simulink model "pfb_fft_d3a"  (R2021a)
settings: Solver=VariableStepAuto  StartTime=0.0  StopTime=100.0  RelTol=1e-3
undefined symbols (not defined in the file): i, pfb_coeff_gen_calc
libraries: xbsIndex_r4 x11529, casper_library_misc x39, casper_library_delays x39, xbsReplacements_r4 x2
(part 3 of 118)

== system pfb_fft_d3a/fft_wideband_real/del_4x_pol0 ==
  d : Inport
  q : Outport  VectorParamsAs1DForOutWhenUnconnected=off
  wires:
  d/1 -> q/1

== system pfb_fft_d3a/fft_wideband_real/del_4x_pol1 ==
  d : Inport
  q : Outport  VectorParamsAs1DForOutWhenUnconnected=off
  wires:
  d/1 -> q/1

== system pfb_fft_d3a/fft_wideband_real/del_4x_pol2 ==
  d : Inport
  q : Outport  VectorParamsAs1DForOutWhenUnconnected=off
  wires:
  d/1 -> q/1

== system pfb_fft_d3a/fft_wideband_real/del_4x_pol3 ==
  d : Inport
  q : Outport  VectorParamsAs1DForOutWhenUnconnected=off
  wires:
  d/1 -> q/1

== system pfb_fft_d3a/fft_wideband_real/del_4x_pol4 ==
  d : Inport
  q : Outport  VectorParamsAs1DForOutWhenUnconnected=off
  wires:
  d/1 -> q/1

== system pfb_fft_d3a/fft_wideband_real/del_4x_pol5 ==
  d : Inport
  q : Outport  VectorParamsAs1DForOutWhenUnconnected=off
  wires:
  d/1 -> q/1

== system pfb_fft_d3a/fft_wideband_real/del_4x_pol6 ==
  d : Inport
  q : Outport  VectorParamsAs1DForOutWhenUnconnected=off
  wires:
  d/1 -> q/1

== system pfb_fft_d3a/fft_wideband_real/del_4x_pol7 ==
  d : Inport
  q : Outport  VectorParamsAs1DForOutWhenUnconnected=off
  wires:
  d/1 -> q/1

== system pfb_fft_d3a/fft_wideband_real/del_direct1 ==
  d : Inport
  q : Outport  VectorParamsAs1DForOutWhenUnconnected=off
  wires:
  d/1 -> q/1

== system pfb_fft_d3a/fft_wideband_real/del_direct2 ==
  d : Inport
  q : Outport  VectorParamsAs1DForOutWhenUnconnected=off
  wires:
  d/1 -> q/1

== system pfb_fft_d3a/fft_wideband_real/del_direct3 ==
  d : Inport
  q : Outport  VectorParamsAs1DForOutWhenUnconnected=off
  wires:
  d/1 -> q/1

== system pfb_fft_d3a/fft_wideband_real/del_direct4 ==
  d : Inport
  q : Outport  VectorParamsAs1DForOutWhenUnconnected=off
  wires:
  d/1 -> q/1

== system pfb_fft_d3a/fft_wideband_real/del_sync_4x ==
  d : Inport
  q : Outport  VectorParamsAs1DForOutWhenUnconnected=off
  wires:
  d/1 -> q/1

== system pfb_fft_d3a/fft_wideband_real/fft_biplex_real_4x ==
  sync : Inport
  shift : Inport  Port=2
  pol0_in : Inport  Port=3
  pol1_in : Inport  Port=4
  pol2_in : Inport  Port=5
  pol3_in : Inport  Port=6
  pol4_in : Inport  Port=7
  pol5_in : Inport  Port=8
  pol6_in : Inport  Port=9
  pol7_in : Inport  Port=10
  bi_real_unscr_4x : Subsystem  AncestorBlock=casper_library_ffts_internal/bi_real_unscr_4x  mask(bi_real_unscr_4x){n_inputs=2, FFTSize=11, n_bits=18, bin_pt=17, floating_point=off, float_type=single, exp_width=8, frac_width=24, add_latency=add_latency, conv_latency=conv_latency, bram_latency=bram_latency, bram_map=on, bram_delays=on, dsp48_adders=off, async=off}
      mask prompts: n_inputs "Number simultaneous inputs (2*?)"; FFTSize "Size of FFT (2^?):"; n_bits "Sample Bit Width"; bin_pt "Sample binary point"; floating_point "floating point"; float_type "float type"; exp_width "exponent width"; frac_width "fraction width"; add_latency "Add Latency"; conv_latency "Convert Latency"; bram_latency "BRAM Latency"; bram_map "Use BlockRAM for Map"; bram_delays "Use BlockRAM for Delays"; dsp48_adders "Use DSP48s for adders"; async "Asynchonrous operation"
      mask help: FFT internal block.
      mask init:
      | bi_real_unscr_4x_init(gcb, ...
      |     'n_inputs', n_inputs, ...
      |     'FFTSize', FFTSize, ...
      |     'n_bits', n_bits, ...
      |     'bin_pt', bin_pt, ...
      |     'floating_point', floating_point, ...
      |     'float_type', float_type, ...
      |     'exp_width', exp_width, ...
      |     'frac_width', frac_width, ...    
      |     'add_latency', add_latency, ...
      |     'conv_latency', conv_latency, ...
      |     'bram_latency', bram_latency, ...
      |     'bram_map', bram_map, ...
      |     'bram_delays', bram_delays, ...
      |     'dsp48_adders', dsp48_adders, ...
      |     'async', async);
      mask Callback floating_point:
      | onoff = get_param(gcb, 'floating_point');
      | if strcmp(onoff,'on')
      |     enable_fixpt = 'off';
      |     set_param_state(gcb, 'float_type', 'on')
      | 
      |     f_type = get_param(gcb, 'float_type');
      |     if strcmp(f_type,'custom')
      |         set_param_state(gcb, 'exp_width', 'on')
      |         set_param_state(gcb, 'frac_width', 'on')
      |     else
      |         set_param_state(gcb, 'exp_width', 'off')
      |         set_param_state(gcb, 'frac_width', 'off')
      |     end
      | 
      | 
      | else
      |     enable_fixpt = 'on';
      |     set_param_state(gcb, 'float_type', 'off')
      |     set_param_state(gcb, 'exp_width', 'off')
      |     set_param_state(gcb, 'frac_width', 'off')
      | end
      | 
      | set_param_state(gcb, 'n_bits', enable_fixpt)
      | set_param_state(gcb, 'bin_pt', enable_fixpt)
      mask TypeOptions float_type: single | custom
      mask Callback float_type:
      | f_type = get_param(gcb, 'float_type');
      | if strcmp(f_type,'custom')
      |     set_param_state(gcb, 'exp_width', 'on')
      |     set_param_state(gcb, 'frac_width', 'on')
      | else
      |     set_param_state(gcb, 'exp_width', 'off')
      |     set_param_state(gcb, 'frac_width', 'off')
      | end
      mask DialogControl ParameterTabVar0 Prompt: Basic
      mask DialogControl ParameterTabVar01 Prompt: Latency
      mask DialogControl ParameterTabVar012 Prompt: Implementation
  biplex_core : Subsystem  AncestorBlock=casper_library_ffts/biplex_core  mask(biplex_core){n_inputs=2, FFTSize=11, input_bit_width=18, bin_pt_in=17, coeff_bit_width=18, floating_point=off, float_type=single, exp_width=8, frac_width=24, add_latency=1, mult_latency=2, bram_latency=2, conv_latency=1, add_pipe_latency=0, mult_pipe_latency=0, quantization=Round  (unbiased: Even Values), overflow=Wrap, delays_bit_limit=9, coeffs_bit_limit=9, coeff_sharing=on, coeff_decimation=on, max_fanout=4, mult_spec=[2 2 2 2 2 2 2 2 2 2 2], bitgrowth=off, max_bits=18, hardcode_shifts=off, shift_schedule=[1 1 1 1 1 1 1 1 1 1 1], dsp48_adders=off, async=off}
      mask prompts: n_inputs "Number inputs (2*?)"; FFTSize "Size of FFT: (2^? pts)"; input_bit_width "Input Bit Width"; bin_pt_in "Input binary point"; coeff_bit_width "Coefficient Bit Width"; floating_point "floating point"; float_type "float type"; exp_width "exponent width"; frac_width "fraction width"; add_latency "Add Latency"; mult_latency "Mult Latency"; bram_latency "BRAM Latency"; conv_latency "Convert latency"; add_pipe_latency "Add Interface Pipeline Latency"; mult_pipe_latency "CMult Pipeline Latency"; quantization "Quantization Behavior"; overflow "Overflow Behavior"; delays_bit_limit "Number bits above which to implent stage's delays in BRAM (2^? bits)"; coeffs_bit_limit "Number bits above which to store stage's coefficients in BRAM (2^? bits)"; coeff_sharing "BRAM sharing in coeff storage"; coeff_decimation "Store a fraction of coeff factors where useful"; max_fanout "Maximum fanout"; mult_spec "Multiplier impl. (0=core, 1=embedded, 2=behavioural) (left=1st stage, or just one value)"; bitgrowth "Bit growth instead of shift"; max_bits "Maximum number of bits"; hardcode_shifts "Hardcode shift schedule"; shift_schedule "Shift schedule"; dsp48_adders "Use DSP48s for adders"; async "Asynchronous operation"
      mask help: FFT internal block.
      mask init:
      | biplex_core_init(gcb, ...
      |     'n_inputs', n_inputs, ...
      |     'FFTSize', FFTSize,...
      |     'input_bit_width', input_bit_width,...
      |     'bin_pt_in', bin_pt_in,...
      |     'coeff_bit_width', coeff_bit_width,...
      |     'floating_point', floating_point, ...
      |     'float_type', float_type, ...
      |     'exp_width', exp_width, ...
      |     'frac_width', frac_width, ...       
      |     'async', async, ...
      |     'add_latency', add_latency,...
      |     'mult_latency', mult_latency,...
      |     'bram_latency', bram_latency,...
      |     'conv_latency', conv_latency, ...
      |     'add_pipe_latency', add_pipe_latency, ...
      |     'mult_pipe_latency', mult_pipe_latency, ...        
      |     'quantization', quantization,...
      |     'overflow', overflow,...
      |     'delays_bit_limit', delays_bit_limit, ...
      |     'coeffs_bit_limit', coeffs_bit_limit, ...
      |     'coeff_sharing', coeff_sharing, ...
      |     'coeff_decimation', coeff_decimation, ...
      |     'max_fanout', max_fanout, ...
      |     'mult_spec', mult_spec, ...
      |     'bitgrowth', bitgrowth, ...
      |     'max_bits', max_bits, ...
      |     'hardcode_shifts', hardcode_shifts, ...
      |     'shift_schedule', shift_schedule, ...
      |     'dsp48_adders', dsp48_adders);
      settings: AttributesFormatString=11 stages
      mask Callback floating_point:
      | onoff = get_param(gcb, 'floating_point');
      | if strcmp(onoff,'on')
      |     enable_fixpt = 'off';
      |     set_param_state(gcb, 'float_type', 'on')
      | 
      |     f_type = get_param(gcb, 'float_type');
      |     if strcmp(f_type,'custom')
      |         set_param_state(gcb, 'exp_width', 'on')
      |         set_param_state(gcb, 'frac_width', 'on')
      |     else
      |         set_param_state(gcb, 'exp_width', 'off')
      |         set_param_state(gcb, 'frac_width', 'off')
      |     end
      | 
      | 
      | else
      |     enable_fixpt = 'on';
      |     set_param_state(gcb, 'float_type', 'off')
      |     set_param_state(gcb, 'exp_width', 'off')
      |     set_param_state(gcb, 'frac_width', 'off')
      | end
      | 
      | set_param_state(gcb, 'input_bit_width', enable_fixpt)
      | set_param_state(gcb, 'bin_pt_in', enable_fixpt)
      | set_param_state(gcb, 'coeff_bit_width', enable_fixpt)
      mask TypeOptions float_type: single | custom
      mask Callback float_type:
      | f_type = get_param(gcb, 'float_type');
      | if strcmp(f_type,'custom')
      |     set_param_state(gcb, 'exp_width', 'on')
      |     set_param_state(gcb, 'frac_width', 'on')
      | else
      |     set_param_state(gcb, 'exp_width', 'off')
      |     set_param_state(gcb, 'frac_width', 'off')
      | end
      mask TypeOptions quantization: Truncate | Round  (unbiased: +/- Inf) | Round  (unbiased: Even Values)
      mask TypeOptions overflow: Wrap | Saturate | Error
      mask Callback hardcode_shifts:
      | hardcode_shifts = get_param(gcb, 'hardcode_shifts');
      | set_param_state(gcb, 'shift_schedule', hardcode_shifts);
      mask Callback dsp48_adders: fft_callback_dsp48_adders(gcb);
      mask DialogControl ParameterTabVar0 Prompt: Basic
      mask DialogControl ParameterTabVar01 Prompt: Latency
      mask DialogControl ParameterTabVar012 Prompt: Implementation
  even_bussify : Subsystem  AncestorBlock=casper_library_flow_control/bus_create  mask(bus_create){inputNum=2}
      mask prompts: inputNum "Number of inputs:"
      mask init:
      | bus_create_init(gcb,...
      |     'inputNum', inputNum);
  odd_bussify : Subsystem  AncestorBlock=casper_library_flow_control/bus_create  mask(bus_create){inputNum=2}
      mask prompts: inputNum "Number of inputs:"
      mask init:
      | bus_create_init(gcb,...
      |     'inputNum', inputNum);
  pol0_debus : Subsystem  AncestorBlock=casper_library_flow_control/bus_expand  mask(bus_expand){mode=divisions of equal size, outputNum=2, outputWidth=36, outputBinaryPt=0, outputArithmeticType=0, show_format=off, outputToWorkspace=off, variablePrefix=out, outputToModelAsWell=on}
      mask prompts: outputNum "Number of outputs:"; outputWidth "Output width:"; outputBinaryPt "Output binary point position:"; outputArithmeticType "Output arithmetic type (ufix=0, fix=1, bool=2):"; show_format "Print format string?"; outputToWorkspace "Output to workspace?"; variablePrefix "Variable name prefix:"; outputToModelAsWell "Output to model as well?"
      mask help:
      | Expands a 'bus' made using a bus_create or Xilinx
      | concat block.
      | The input will be divided into the specified number
      | of outputs with the specified arithmetic types.
      | Divisions are made from most significant bit.
      mask init:
      | bus_expand_init(gcb,...
      |     'mode', mode, ...
      |     'outputNum', outputNum, ...
      |     'outputWidth', outputWidth, ...
      |     'outputBinaryPt', outputBinaryPt, ...
      |     'outputArithmeticType', outputArithmeticType, ...
      |     'show_format', show_format, ...
      |     'outputToWorkspace', outputToWorkspace, ...
      |     'variablePrefix', variablePrefix, ...
      |     'outputToModelAsWell', outputToModelAsWell);
      settings: AttributesFormatString=2 outputs
      mask TypeOptions mode: divisions of equal size | divisions of arbitrary size
      mask Callback mode: %bus_expand_callback();
      mask Callback outputWidth: %bus_expand_callback();
      mask Callback outputToWorkspace: %bus_expand_callback();
  pol1_debus : Subsystem  AncestorBlock=casper_library_flow_control/bus_expand  mask(bus_expand){mode=divisions of equal size, outputNum=2, outputWidth=36, outputBinaryPt=0, outputArithmeticType=0, show_format=off, outputToWorkspace=off, variablePrefix=out, outputToModelAsWell=on}
      mask prompts: outputNum "Number of outputs:"; outputWidth "Output width:"; outputBinaryPt "Output binary point position:"; outputArithmeticType "Output arithmetic type (ufix=0, fix=1, bool=2):"; show_format "Print format string?"; outputToWorkspace "Output to workspace?"; variablePrefix "Variable name prefix:"; outputToModelAsWell "Output to model as well?"
      mask help:
      | Expands a 'bus' made using a bus_create or Xilinx
      | concat block.
      | The input will be divided into the specified number
      | of outputs with the specified arithmetic types.
      | Divisions are made from most significant bit.
      mask init: same as pfb_fft_d3a/fft_wideband_real/fft_biplex_real_4x/pol0_debus
      settings: AttributesFormatString=2 outputs
      mask TypeOptions mode: divisions of equal size | divisions of arbitrary size
      mask Callback mode: %bus_expand_callback();
      mask Callback outputWidth: %bus_expand_callback();
      mask Callback outputToWorkspace: %bus_expand_callback();
  pol2_debus : Subsystem  AncestorBlock=casper_library_flow_control/bus_expand  mask(bus_expand){mode=divisions of equal size, outputNum=2, outputWidth=36, outputBinaryPt=0, outputArithmeticType=0, show_format=off, outputToWorkspace=off, variablePrefix=out, outputToModelAsWell=on}
      mask prompts: outputNum "Number of outputs:"; outputWidth "Output width:"; outputBinaryPt "Output binary point position:"; outputArithmeticType "Output arithmetic type (ufix=0, fix=1, bool=2):"; show_format "Print format string?"; outputToWorkspace "Output to workspace?"; variablePrefix "Variable name prefix:"; outputToModelAsWell "Output to model as well?"
      mask help:
      | Expands a 'bus' made using a bus_create or Xilinx
      | concat block.
      | The input will be divided into the specified number
      | of outputs with the specified arithmetic types.
      | Divisions are made from most significant bit.
      mask init: same as pfb_fft_d3a/fft_wideband_real/fft_biplex_real_4x/pol0_debus
      settings: AttributesFormatString=2 outputs
      mask TypeOptions mode: divisions of equal size | divisions of arbitrary size
      mask Callback mode: %bus_expand_callback();
      mask Callback outputWidth: %bus_expand_callback();
      mask Callback outputToWorkspace: %bus_expand_callback();
  pol3_debus : Subsystem  AncestorBlock=casper_library_flow_control/bus_expand  mask(bus_expand){mode=divisions of equal size, outputNum=2, outputWidth=36, outputBinaryPt=0, outputArithmeticType=0, show_format=off, outputToWorkspace=off, variablePrefix=out, outputToModelAsWell=on}
      mask prompts: outputNum "Number of outputs:"; outputWidth "Output width:"; outputBinaryPt "Output binary point position:"; outputArithmeticType "Output arithmetic type (ufix=0, fix=1, bool=2):"; show_format "Print format string?"; outputToWorkspace "Output to workspace?"; variablePrefix "Variable name prefix:"; outputToModelAsWell "Output to model as well?"
      mask help:
      | Expands a 'bus' made using a bus_create or Xilinx
      | concat block.
      | The input will be divided into the specified number
      | of outputs with the specified arithmetic types.
      | Divisions are made from most significant bit.
      mask init: same as pfb_fft_d3a/fft_wideband_real/fft_biplex_real_4x/pol0_debus
      settings: AttributesFormatString=2 outputs
      mask TypeOptions mode: divisions of equal size | divisions of arbitrary size
      mask Callback mode: %bus_expand_callback();
      mask Callback outputWidth: %bus_expand_callback();
      mask Callback outputToWorkspace: %bus_expand_callback();
  ri_to_c0 : Subsystem  AncestorBlock=casper_library_misc/ri_to_c  mask(ri_to_c){}
      mask help:
      | Concatenates real and imaginary inputs into a complex output.
      | Useful for simplifying interconnects.
      | See also: Complex to Real-Imag (c_to_ri)
      mask Help: eval('xlWeb(''http://casper.berkeley.edu/wiki/Ri_to_c'')')
  ri_to_c1 : Subsystem  AncestorBlock=casper_library_misc/ri_to_c  mask(ri_to_c){}
      mask help:
      | Concatenates real and imaginary inputs into a complex output.
      | Useful for simplifying interconnects.
      | See also: Complex to Real-Imag (c_to_ri)
      mask Help: eval('xlWeb(''http://casper.berkeley.edu/wiki/Ri_to_c'')')
  ri_to_c2 : Subsystem  AncestorBlock=casper_library_misc/ri_to_c  mask(ri_to_c){}
      mask help:
      | Concatenates real and imaginary inputs into a complex output.
      | Useful for simplifying interconnects.
      | See also: Complex to Real-Imag (c_to_ri)
      mask Help: eval('xlWeb(''http://casper.berkeley.edu/wiki/Ri_to_c'')')
  ri_to_c3 : Subsystem  AncestorBlock=casper_library_misc/ri_to_c  mask(ri_to_c){}
      mask help:
      | Concatenates real and imaginary inputs into a complex output.
      | Useful for simplifying interconnects.
      | See also: Complex to Real-Imag (c_to_ri)
      mask Help: eval('xlWeb(''http://casper.berkeley.edu/wiki/Ri_to_c'')')
  sync_out : Outport
  pol0_out : Outport  Port=2
  pol1_out : Outport  Port=3
  pol2_out : Outport  Port=4
  pol3_out : Outport  Port=5
  pol4_out : Outport  Port=6
  pol5_out : Outport  Port=7
  pol6_out : Outport  Port=8
  pol7_out : Outport  Port=9
  of : Outport  Port=10
  wires:
  pol0_debus/1(msb_out2) -> pol0_out/1
  pol0_in/1 -> ri_to_c0/1(re)
  pol1_in/1 -> ri_to_c0/2(im)
  ri_to_c0/1(c) -> even_bussify/1(in1)
  pol1_debus/1(msb_out2) -> pol1_out/1
  pol2_debus/1(msb_out2) -> pol2_out/1
  pol2_in/1 -> ri_to_c1/1(re)
  pol3_in/1 -> ri_to_c1/2(im)
  ri_to_c1/1(c) -> odd_bussify/1(in1)
  pol3_debus/1(msb_out2) -> pol3_out/1
  pol0_debus/2(lsb_out1) -> pol4_out/1
  pol4_in/1 -> ri_to_c2/1(re)
  pol5_in/1 -> ri_to_c2/2(im)
  ri_to_c2/1(c) -> even_bussify/2(in2)
  pol1_debus/2(lsb_out1) -> pol5_out/1
  pol2_debus/2(lsb_out1) -> pol6_out/1
  pol6_in/1 -> ri_to_c3/1(re)
  pol7_in/1 -> ri_to_c3/2(im)
  ri_to_c3/1(c) -> odd_bussify/2(in2)
  pol3_debus/2(lsb_out1) -> pol7_out/1
  sync/1 -> biplex_core/1(sync)
  shift/1 -> biplex_core/2(shift)
  even_bussify/1(bus_out) -> biplex_core/3(pol1)
  odd_bussify/1(bus_out) -> biplex_core/4(pol2)
  biplex_core/4(of) -> of/1
  biplex_core/1(sync_out) -> bi_real_unscr_4x/1(sync)
  biplex_core/2(out1) -> bi_real_unscr_4x/2(even)
  biplex_core/3(out2) -> bi_real_unscr_4x/3(odd)
  bi_real_unscr_4x/1(sync_out) -> sync_out/1
  bi_real_unscr_4x/2(pol1_out) -> pol0_debus/1(bus_in)
  bi_real_unscr_4x/3(pol2_out) -> pol1_debus/1(bus_in)
  bi_real_unscr_4x/4(pol3_out) -> pol2_debus/1(bus_in)
  bi_real_unscr_4x/5(pol4_out) -> pol3_debus/1(bus_in)
